simulink model "Suspensie_Activa_Regresie"  (R2022b)
settings: Solver=FixedStepAuto  StartTime=0.0  StopTime=Tfin  FixedStep=Ts  RelTol=1e-3
values from neighbouring files (symbols this model uses):
  a1 = [      2*p(1)*p(2),      p(1)*p(5)/p(6) ... (first row only)    [Setup_Suspensie_Activa_Regresie.m]
  a2 = [      p(1)*p(6)/p(5),      p(1)*p(5)*p(3) ... (first row only)    [Setup_Suspensie_Activa_Regresie.m]
  b0 = p(4)/p(6)    [Setup_Suspensie_Activa_Regresie.m]
  t1 = round(0.33*Tfin/Ts)*Ts    [Setup_Suspensie_Activa_Regresie.m]
  t2 = 2*t1    [Setup_Suspensie_Activa_Regresie.m]
  Ts = 2e-3    (= 0.002)    [Setup_Suspensie_Activa_Regresie.m]
  u1 = 0    [Setup_Suspensie_Activa_Regresie.m]
  u2 = 600    [Setup_Suspensie_Activa_Regresie.m]
  u_op_region = -350 + 700*r(7)    [Setup_Suspensie_Activa_Regresie.m]
  umax = 3000    [Setup_Suspensie_Activa_Regresie.m]
  umin = -3000    [Setup_Suspensie_Activa_Regresie.m]
  whtn_pow_in = sigma_u^2*whtn_Ts_in/2    [Setup_Suspensie_Activa_Regresie.m]
  whtn_pow_out = sigma_y^2*whtn_Ts_out    [Setup_Suspensie_Activa_Regresie.m]
  whtn_seed_in = 41000 + 2*student_id    (= 41088)    [Setup_Suspensie_Activa_Regresie.m]
  whtn_seed_out = 41001 + 2*student_id    (= 41089)    [Setup_Suspensie_Activa_Regresie.m]
  whtn_Ts_in = 3*Ts    (= 0.006)    [Setup_Suspensie_Activa_Regresie.m]
  whtn_Ts_out = 3*Ts    (= 0.006)    [Setup_Suspensie_Activa_Regresie.m]
  x0_slx = [ ... (first row only)    [Setup_Suspensie_Activa_Regresie.m]
  ymax = 35    [Setup_Suspensie_Activa_Regresie.m]
  ymin = -35    [Setup_Suspensie_Activa_Regresie.m]
libraries: simulink x2
settings Model: Creator=mircea  LastModifiedBy=mircea
settings OptimizationCC: ReuseModelBlockBuffer=on
settings RTWCC: GPUComputeCapability=5.0
settings ConfigComp: CovBoundaryAbsTol=1.0e-5

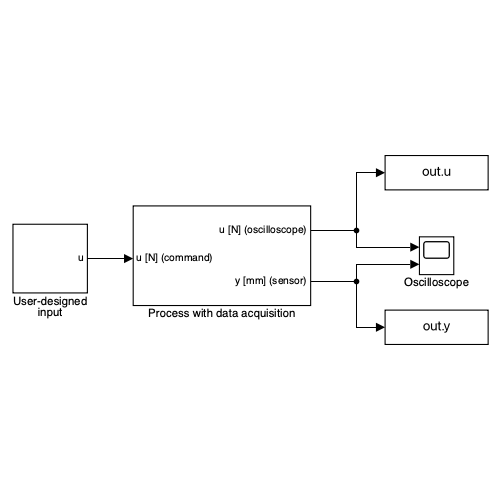
[thumbnail: Simulink's stored preview of the top-level diagram]
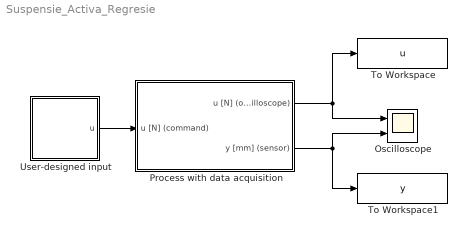
== system Suspensie_Activa_Regresie ==
  Oscilloscope : Scope  NumInputPorts=2
  Process with data acquisition : Subsystem
  To Workspace : ToWorkspace  VariableName=u  SampleTime=Ts
  To Workspace1 : ToWorkspace  VariableName=y  SampleTime=Ts
  User-designed input : Subsystem
  wires:
  Process with data acquisition/1(u [N] (oscilloscope)) -> Oscilloscope/1, To Workspace/1
  Process with data acquisition/2(y [mm] (sensor)) -> Oscilloscope/2, To Workspace1/1
  User-designed input/1(u) -> Process with data acquisition/1(u [N] (command))

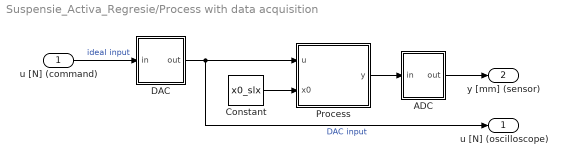
== system Suspensie_Activa_Regresie/Process with data acquisition ==
  u [N] (command) : Inport
  ADC : Subsystem
  Constant : Constant  Value=x0_slx
  DAC : Subsystem
  Process : Subsystem
  u [N] (oscilloscope) : Outport
  y [mm] (sensor) : Outport  Port=2
  wires:
  Constant/1 -> Process/2(x0)
  u [N] (command)/1 -> DAC/1(in)  "ideal input"
  Process/1(y) -> ADC/1(in)
  ADC/1(out) -> y [mm] (sensor)/1
  DAC/1(out) -> Process/1(u), u [N] (oscilloscope)/1  "DAC input"

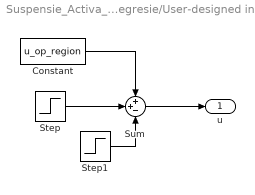
== system Suspensie_Activa_Regresie/User-designed input ==
  Constant : Constant  Value=u_op_region
  Step : Step  Time=t1  Before=u1  After=u2  SampleTime=0
  Step1 : Step  Time=t2  Before=u1  After=u2  SampleTime=0
  Sum : Sum  Inputs=++-
  u : Outport
  wires:
  Constant/1 -> Sum/1
  Sum/1 -> u/1
  Step/1 -> Sum/2
  Step1/1 -> Sum/3

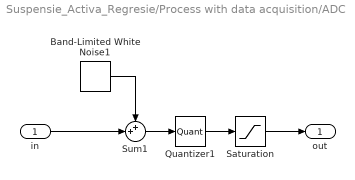
== system Suspensie_Activa_Regresie/Process with data acquisition/ADC ==
  in : Inport
  Band-Limited White Noise1 : simulink/Sources/Band-Limited White Noise  Cov=[whtn_pow_out]  Ts=whtn_Ts_out  seed=[whtn_seed_out]
  Quantizer1 : Quantizer  QuantizationInterval=q_out
  Saturation : Saturate  UpperLimit=ymax  LowerLimit=ymin
  Sum1 : Sum  Inputs=++|
  out : Outport
  wires:
  Quantizer1/1 -> Saturation/1
  Sum1/1 -> Quantizer1/1
  in/1 -> Sum1/2
  Band-Limited White Noise1/1 -> Sum1/1
  Saturation/1 -> out/1

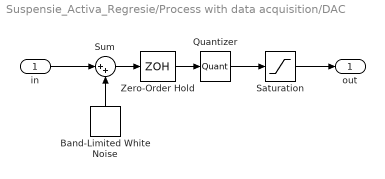
== system Suspensie_Activa_Regresie/Process with data acquisition/DAC ==
  in : Inport
  Band-Limited White Noise : simulink/Sources/Band-Limited White Noise  Cov=[whtn_pow_in]  Ts=whtn_Ts_in  seed=[whtn_seed_in]
  Quantizer : Quantizer  QuantizationInterval=q_in
  Saturation : Saturate  UpperLimit=umax  LowerLimit=umin
  Sum : Sum  Inputs=|++
  Zero-Order Hold : ZeroOrderHold  SampleTime=-1
  out : Outport
  wires:
  Quantizer/1 -> Saturation/1
  Sum/1 -> Zero-Order Hold/1
  in/1 -> Sum/1
  Band-Limited White Noise/1 -> Sum/2
  Zero-Order Hold/1 -> Quantizer/1
  Saturation/1 -> out/1

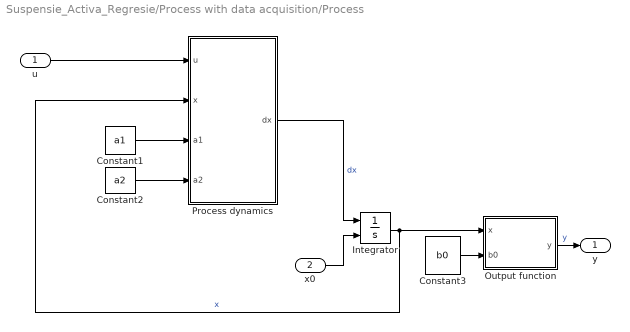
== system Suspensie_Activa_Regresie/Process with data acquisition/Process ==
  u : Inport
  x0 : Inport  Port=2
  Constant1 : Constant  Value=a1
  Constant2 : Constant  Value=a2
  Constant3 : Constant  Value=b0
  Integrator : Integrator  InitialConditionSource=external
  Output function : MATLAB Function  TreatAsAtomicUnit=on
  Process dynamics : MATLAB Function  TreatAsAtomicUnit=on
  y : Outport
  wires:
  u/1 -> Process dynamics/1(u)
  Process dynamics/1(dx) -> Integrator/1  "dx"
  Integrator/1 -> Output function/1(x), Process dynamics/2(x)  "x"
  Output function/1(y) -> y/1  "y"
  x0/1 -> Integrator/2
  Constant2/1 -> Process dynamics/4(a2)
  Constant1/1 -> Process dynamics/3(a1)
  Constant3/1 -> Output function/2(b0)

== matlab function Suspensie_Activa_Regresie/Process with data acquisition/Process/Process dynamics ==
  data: u input; dx output; x input; a1 input; a2 input
function dx = fcn(u,x,a1,a2)

dx = [
    -a1(1)*x(1) - a1(2)*x(2) + a2(2)*u;
     a2(1)*x(1)
];

end

== matlab function Suspensie_Activa_Regresie/Process with data acquisition/Process/Output function ==
  data: y output; x input; b0 input
function y = fcn(x,b0)

y = b0*x(2);

end
